simulink model "sf_cdplayer_STT"  (R2025b)
settings: Solver=FixedStepDiscrete  StartTime=0.0  StopTime=inf  FixedStep=1  RelTol=1e-3  EnableMultiTasking=on
PreLoadFcn:
  | defaultRadioRequestMode = RadioRequestMode.OFF;
  | defaultCdRequestMode = CdRequestMode.EMPTY;
StartFcn:
  | clear sfcdplayerhelper_STT;
  | sfcdplayergui_STT;
StopFcn:
  | delete(sfcdplayergui_STT);
model workspace (MATLAB code in the model file):
  | Ts = 0.01;  % setup system sample rate
undefined symbols (not defined in the file or in its folder): CdRequestMode, RadioRequestMode
settings Model: Creator=The MathWorks, Inc.  LastModifiedBy=The MathWorks, Inc.
settings SolverCC: AlgebraicLoopSolver=TrustRegion  MaxZcPerStep=1.0
settings DataIOCC: LimitDataPoints=on  SaveFormat=Array  SaveOutput=off  SaveTime=off  ReturnWorkspaceOutputs=off
settings OptimizationCC: ReuseModelBlockBuffer=off  ExpressionDepthLimit=2147483647.0  StateBitsets=on  DataBitsets=on  ZeroExternalMemoryAtStartup=off  ZeroInternalMemoryAtStartup=off  InitFltsAndDblsToZero=on  EfficientFloat2IntCast=on  EfficientMapNaN2IntZero=off  LifeSpan=1  EfficientTunableParamExpr=on
settings DebuggingCC: UnderspecifiedInitializationDetection=Classic  MergeDetectMultiDrivingBlocksExec=none  FcnCallInpInsideContextMsg=warning  UnconnectedInputMsg=warning  UnconnectedOutputMsg=warning  UnconnectedLineMsg=warning  AllowSymbolicDim=off  StateNameClashWarn=warning  SFUnexpectedBacktrackingDiag=warning  SFNoUnconditionalDefaultTransitionDiag=warning  SFExecutionAtInitializationDiag=none  ArithmeticOperatorsInVariantConditions=warning
settings HardwareCC: ProdBitPerPointer=32.0  ProdBitPerSizeT=32.0  ProdBitPerPtrDiffT=32.0  ProdLargestAtomicFloat=None  ProdWordSize=32.0  ProdHWDeviceType=NEC->V850
settings ModelReferenceCC: EnableRefExpFcnMdlSchedulingChecks=on  ModelReferenceNumInstancesAllowed=Single  PropagateSignalLabelsOutOfModel=off
settings SFSimCC: SimUseLocalCustomCode=off  SimParseCustomCode=off  CustomCodeUndefinedFunction=UseInterfaceOnly
settings RTWCC: SystemTargetFile=ert.tlc  GenCodeOnly=on  TemplateMakefile=ert_default_tmf  GenerateReport=on  RTWUseLocalCustomCode=off  IncludeHyperlinkInReport=on  LaunchReport=on  GenerateTraceInfo=on  GenerateTraceReport=on  GenerateTraceReportSl=on  GenerateTraceReportSf=on  GenerateTraceReportEml=on  GPUComputeCapability=3.5  DLArmComputeVersion=19.05  Description=Real-Time Workshop Embedded Coder (no auto configuration)
settings CodeAppCC: IgnoreCustomStorageClasses=off  CustomSymbolStrType=$N$R$M  CustomSymbolStrModelFcn=$N  StateflowObjectComments=on  InternalIdentifier=Classic
settings ERTTargetCC: InlinedParameterPlacement=Hierarchical  ERTCustomFileTemplate=example_file_process.tlc  ConvertIfToSwitch=off  SuppressUnreachableDefaultCases=off  EnableUserReplacementTypes=on  DynamicArrayContainerType=coder::array  MultiwordLength=2048.0  GenerateSampleERTMain=on  IncludeMdlTerminateFcn=off  SupportAbsoluteTime=off  SubcomponentCodeInterfacePackaging=Nonreusable function  SupportNonFinite=off  SupportComplex=off  SupportContinuousTime=on
settings ConfigComp: CovMetricSettings=dw  CovSaveCumulativeToWorkspaceVar=on  CovSaveSingleToWorkspaceVar=on  CovExternalEMLEnable=off  CovSFcnEnable=off  DVMaxProcessTime=600.0  DVParameters=on  DVModelCoverageObjectives=MCDC  DVMaxTestCaseSteps=500.0  DVTestSuiteOptimization=Auto  DVAbsoluteTolerance=1.0e-5  DVDefectChecker=off  DVDetectActiveLogic=on  DVMaxViolationSteps=20.0  DVSaveHarnessModel=on  DVModelReferenceHarness=on  DVHarnessSource=Signal Editor  DVSaveReport=on  DVActiveTab=0.0

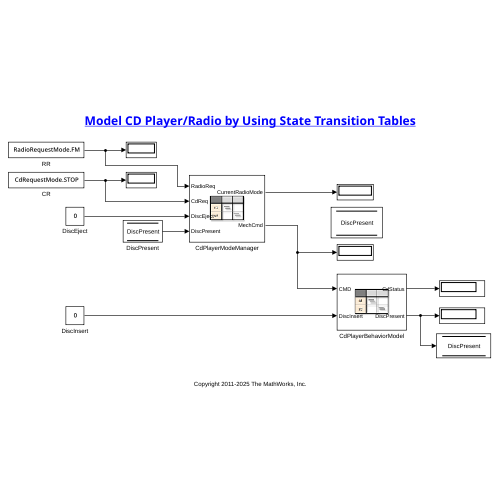
[thumbnail: Simulink's stored preview of the top-level diagram]
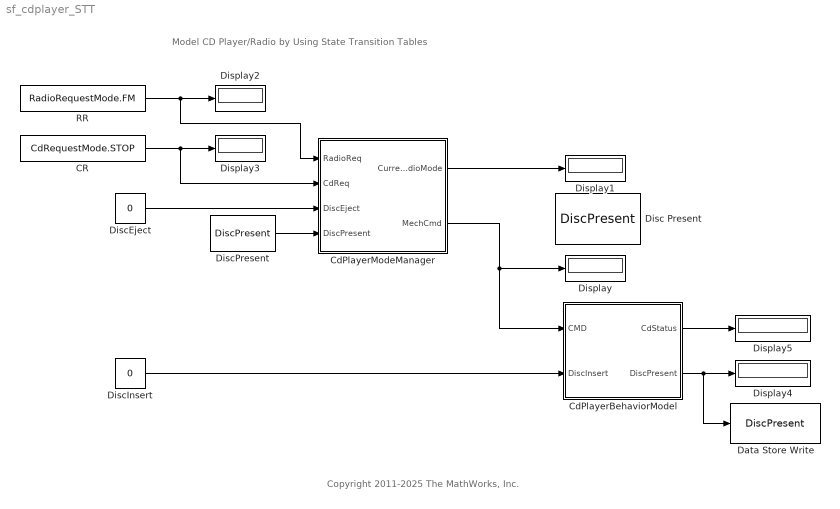
== system sf_cdplayer_STT ==
  note: Copyright 2011-2025 The MathWorks, Inc.
  note: Model CD Player/Radio by Using State Transition Tables
  CR : Constant  Value=CdRequestMode.STOP  OutDataTypeStr=Enum: CdRequestMode
  CdPlayerBehaviorModel : State Transition Table  TreatAsAtomicUnit=on
  CdPlayerModeManager : State Transition Table  TreatAsAtomicUnit=on
  Data Store Write : DataStoreWrite  DataStoreName=DiscPresent  IndexOptions=Index vector (dialog)  Indices=1  OutputSizes=1
  Disc Present : DataStoreMemory  DataStoreName=DiscPresent  ShowAdditionalParam=off
  DiscEject : Constant  LoadFcn=set_param(gcb,'Value','0');  StartFcn="h1   = add_exec_event_listener(gcb,'PostOutputs',@sfcdplayerhelper_STT);"  StopFcn=set_param(gcb,'Value','0');  Value=0  OutDataTypeStr=boolean
  DiscInsert : Constant  LoadFcn=set_param(gcb,'Value','0');  StartFcn="h2   = add_exec_event_listener(gcb,'PostOutputs',@sfcdplayerhelper_STT);"  StopFcn=set_param(gcb,'Value','0');  Value=0  OutDataTypeStr=boolean
  DiscPresent : DataStoreRead  DataStoreName=DiscPresent  SampleTime=0  IndexOptions=Index vector (dialog)  Indices=1  OutputSizes=1
  Display{,1..5} (6 alike) : Display
  RR : Constant  Value=RadioRequestMode.FM  OutDataTypeStr=Enum: RadioRequestMode
  wires:
  CR/1 -> CdPlayerModeManager/2(CdReq), Display3/1
  DiscPresent/1 -> CdPlayerModeManager/4(DiscPresent)
  CdPlayerModeManager/2(MechCmd) -> Display/1, CdPlayerBehaviorModel/1(CMD)
  CdPlayerModeManager/1(CurrentRadioMode) -> Display1/1
  RR/1 -> CdPlayerModeManager/1(RadioReq), Display2/1
  CdPlayerBehaviorModel/1(CdStatus) -> Display5/1
  CdPlayerBehaviorModel/2(" DiscPresent") -> Data Store Write/1, Display4/1
  DiscInsert/1 -> CdPlayerBehaviorModel/2(DiscInsert)
  DiscEject/1 -> CdPlayerModeManager/3(DiscEject)

== stateflow chart sf_cdplayer_STT/CdPlayerModeManager ==
  state ModeManager
    (history)
    state Standby
      entry:
      CurrentRadioMode = RadioRequestMode.OFF;
      MechCmd = CdRequestMode.STOP;
    state ON
      (history)
      state CDMode
        entry: CurrentRadioMode = RadioRequestMode.CD;
        MechCmd =  CdRequestMode.STOP;
        ex: MechCmd =  CdRequestMode.STOP;
        state Stop
          entry: MechCmd = CdRequestMode.STOP;
        state Play
          state FastForward
            entry: MechCmd = CdRequestMode.FF;
          state Rew
            entry: MechCmd = CdRequestMode.REW;
          state Normal
            entry: MechCmd = CdRequestMode.PLAY;
          Play -> (junction 125) [order 1]
          (junction 125) -> FastForward [order 1] : [CdReq == CdRequestMode.FF && ~in(FastForward)]
          (junction 125) -> (junction 131) [order 2]
          (junction 131) -> Rew [order 1] : [CdReq == CdRequestMode.REW && ~in(Rew)]
          (junction 131) -> (junction 128) [order 2]
          (default) -> Normal
          (junction 128) -> Normal : [CdReq == CdRequestMode.PLAY && ~in(Normal)]
        (default) -> Stop [order 2]
        Stop -> Play : [DiscPresent && CdReq==CdRequestMode.PLAY]
        Play -> Stop [order 1] : [CdReq==CdRequestMode.STOP]
        (default) -> Play [order 1] : [DiscPresent]
      state AMMode
        entry:
        CurrentRadioMode = RadioRequestMode.AM;
        MechCmd = CdRequestMode.STOP;
      state FMMode
        entry:
        CurrentRadioMode = RadioRequestMode.FM;
        MechCmd = CdRequestMode.STOP;
      (default) -> (junction 74)
      ON -> (junction 74) [order 1] : [hasChanged(RadioReq)]
      (junction 74) -> CDMode [order 1] : [RadioReq == RadioRequestMode.CD]
      (junction 74) -> (junction 77) [order 2]
      (junction 77) -> AMMode [order 1] : [RadioReq == RadioRequestMode.AM]
      (junction 77) -> (junction 80) [order 2]
      (junction 80) -> FMMode
    (default) -> Standby
    Standby -> ON : [RadioReq ~= RadioRequestMode.OFF]
    ON -> Standby [order 1] : [RadioReq == RadioRequestMode.OFF]
  state Eject
    entry:
    MechCmd = CdRequestMode.EJECT;
  (default) -> ModeManager
  ModeManager -> Eject : [DiscEject]
  Eject -> ModeManager
  data: RadioReq input Enum: RadioRequestMode =0xFF; CdReq input Enum: CdRequestMode; DiscEject input; CurrentRadioMode output Enum: RadioRequestMode; DiscPresent input boolean; MechCmd output Enum: CdRequestMode

== stateflow chart sf_cdplayer_STT/CdPlayerBehaviorModel ==
  state Empty
    entry: CdStatus = CdRequestMode.EMPTY;
  state Inserting
    entry: CdStatus = CdRequestMode.DISCINSERT;
  state Ejecting
    entry: CdStatus = CdRequestMode.EJECT;
  state DiscPresent
    state STOP
      entry: CdStatus = CdRequestMode.STOP;
    state PLAY
      entry: CdStatus = CdRequestMode.PLAY;
    state REW
      entry: CdStatus = CdRequestMode.REW;
    state FF
      entry: CdStatus = CdRequestMode.FF;
    (default) -> STOP
    DiscPresent -> (junction 78) [order 1]
    (junction 78) -> STOP [order 1] : [CMD == CdRequestMode.STOP]
    (junction 78) -> (junction 71) [order 2]
    (junction 71) -> PLAY [order 1] : [CMD == CdRequestMode.PLAY]
    (junction 71) -> (junction 83) [order 2]
    (junction 83) -> REW [order 1] : [CMD == CdRequestMode.REW]
    (junction 83) -> (junction 86) [order 2]
    (junction 86) -> FF : [CMD == CdRequestMode.FF]
  (default) -> Empty
  (junction 33) -> Empty
  (junction 35) -> (junction 33)
  Empty -> Inserting : [DiscInsert]
  Inserting -> (junction 30) : [after(1/Ts, tick)]
  (junction 30) -> (junction 28)
  Ejecting -> (junction 35) : [after(1/Ts, tick)]
  DiscPresent -> Ejecting [order 1] : [CMD == CdRequestMode.EJECT]
  (junction 28) -> DiscPresent
  data: CMD input Enum: CdRequestMode size=1; CdStatus output Enum: CdRequestMode; DiscInsert input boolean; Ts parameter double size=1; DiscPresent output boolean
